simulink model "lga"  (R2020a)
settings: Solver=ode45  StartTime=0.0  StopTime=0.4  FixedStep=1e-6  MaxStep=0.04  RelTol=1e-3  EnableMultiTasking=on
PreLoadFcn:
  | power_13NodeTestFeeder_init;
values from neighbouring files (symbols this model uses):
  C_601 = [1.03835973183e-08  -3.28956213337e-09  -2.07596127216e-09; -3.28956213337e-09  9.8230300863e-09  -1.22250137004e-09; -2.07596127216e-09  -1.22250137004e-09  9.29377945947e-09]    [bus9.mat]    (also in matlab.mat)
  C_602 = [9.39333329896e-09  -1.78290377777e-09  -2.78635373607e-09; -1.78290377777e-09  8.5370713848e-09  -1.08586207709e-09; -2.78635373607e-09  -1.08586207709e-09  8.94105559107e-09]    [bus9.mat]    (also in matlab.mat)
  C_603 = [0  0  0; 0  7.76272711671e-09  -1.48325331387e-09; 0  -1.48325331387e-09  7.69036927641e-09]    [bus9.mat]    (also in matlab.mat)
  C_604 = [7.69036927641e-09  0  -1.48325331387e-09; 0  0  0; -1.48325331387e-09  0  7.76272711671e-09]    [bus9.mat]    (also in matlab.mat)
  C_605 = [0  0  0; 0  0  0; 0  0  7.44890176838e-09]    [bus9.mat]    (also in matlab.mat)
  C_606 = [1.59697709306e-07  -1.64824237567e-15  -1.64824237567e-15; -1.64824237567e-15  1.59697709306e-07  -1.64824237567e-15; -1.64824237567e-15  -1.64824237567e-15  1.59697709306e-07]    [bus9.mat]    (also in matlab.mat)
  C_607 = [1.46679066902e-07  0  0; 0  0  0; 0  0  0]    [bus9.mat]    (also in matlab.mat)
  ft2km = 0.0003048    [bus9.mat]    (also in matlab.mat)
  L_601 = [0.0016777459142  0.000826923199875  0.000698195470335; 0.000826923199875  0.00172702836123  0.000634408490396; 0.000698195470335  0.000634408490396  0.00170560121035]    [bus9.mat]    (also in matlab.mat)
  L_602 = [0.00194723354262  0.000698195470335  0.000826923199875; 0.000698195470335  0.00197508883877  0.000634408490396; 0.000826923199875  0.000634408490396  0.00199635116541]    [bus9.mat]    (also in matlab.mat)
  L_603 = [0  0  0; 0  0.00222034730427  0.000756708074671; 0  0.000756708074671  0.00223650007955]    [bus9.mat]    (also in matlab.mat)
  L_604 = [0.00223650007955  0  0.000756708074671; 0  0  0; 0.000756708074671  0  0.00222034730427]    [bus9.mat]    (also in matlab.mat)
  L_605 = [0  0  0; 0  0  0; 0  0  0.00222100660122]    [bus9.mat]    (also in matlab.mat)
  L_606 = [0.000735610572263  5.40623499221e-05  2.35698659721e-05; 5.40623499221e-05  0.000666054744009  5.40623499221e-05; 2.35698659721e-05  5.40623499221e-05  0.000735610572263]    [bus9.mat]    (also in matlab.mat)
  L_607 = [0.000844559393295  0  0; 0  0  0; 0  0  0]    [bus9.mat]    (also in matlab.mat)
  R_601 = [0.215305653249  0.0969341469174  0.0981768923907; 0.0969341469174  0.209713298619  0.0953807150757; 0.0981768923907  0.0953807150757  0.212136652292]    [bus9.mat]    (also in matlab.mat)
  R_602 = [0.467645121603  0.0981768923907  0.0969341469174; 0.0981768923907  0.464476120646  0.0953807150757; 0.0969341469174  0.0953807150757  0.462052766973]    [bus9.mat]    (also in matlab.mat)
  R_603 = [0  0  0; 0  0.826052916102  0.128375607392; 0  0.128375607392  0.822573228777]    [bus9.mat]    (also in matlab.mat)
  R_604 = [0.822573228777  0  0.128375607392; 0  0  0; 0.128375607392  0  0.826052916102]    [bus9.mat]    (also in matlab.mat)
  R_605 = [0  0  0; 0  0  0; 0  0  0.825928641555]    [bus9.mat]    (also in matlab.mat)
  R_606 = [0.495979718394  0.198342177539  0.177029092672; 0.198342177539  0.49032522649  0.198342177539; 0.177029092672  0.198342177539  0.495979718394]    [bus9.mat]    (also in matlab.mat)
  R_607 = [0.834192898952  0  0; 0  0  0; 0  0  0]    [bus9.mat]    (also in matlab.mat)
libraries: powerlib x54, powerlib_meascontrol x6
settings Model: Creator=MathWorks  LastModifiedBy=LMS Solution
settings DataIOCC: ExternalInput=getinputstruct(op_IEEE_13_node_5)  InitialState=getstatestruct(op_IEEE_13_node_5)  LimitDataPoints=on  SaveFormat=Array  SignalLoggingSaveFormat=ModelDataLogs  ReturnWorkspaceOutputs=off
settings OptimizationCC: ExpressionDepthLimit=2147483647  LifeSpan=inf
settings DebuggingCC: AlgebraicLoopMsg=none  UnderspecifiedInitializationDetection=Classic  MergeDetectMultiDrivingBlocksExec=none  FcnCallInpInsideContextMsg=warning  UnconnectedInputMsg=none  UnconnectedOutputMsg=none  UnconnectedLineMsg=none  AllowSymbolicDim=off  StateNameClashWarn=warning  SFUnexpectedBacktrackingDiag=warning  SFNoUnconditionalDefaultTransitionDiag=warning  SFExecutionAtInitializationDiag=none  ArithmeticOperatorsInVariantConditions=warning
settings HardwareCC: ProdBitPerPointer=32  ProdBitPerSizeT=32  ProdBitPerPtrDiffT=32  ProdLargestAtomicFloat=None  ProdIntDivRoundTo=Undefined  ProdEndianess=Unspecified  ProdWordSize=32  ProdHWDeviceType=32-bit Generic
settings ModelReferenceCC: PropagateSignalLabelsOutOfModel=off
settings SFSimCC: SimUseLocalCustomCode=off  CustomCodeUndefinedFunction=UseInterfaceOnly
settings RTWCC: RTWUseLocalCustomCode=off
settings CodeAppCC: StateflowObjectComments=on
settings GRTTargetCC: TargetLangStandard=C89/C90 (ANSI)  CombineOutputUpdateFcns=off  GRTInterface=on
settings ConfigComp: CovMetricSettings=dw  CovHtmlReporting=on  CovSaveCumulativeToWorkspaceVar=on  CovSaveSingleToWorkspaceVar=on  CovExternalEMLEnable=off  CovSFcnEnable=off
settings SimscapeCC: SimscapeNormalizeSystem=off

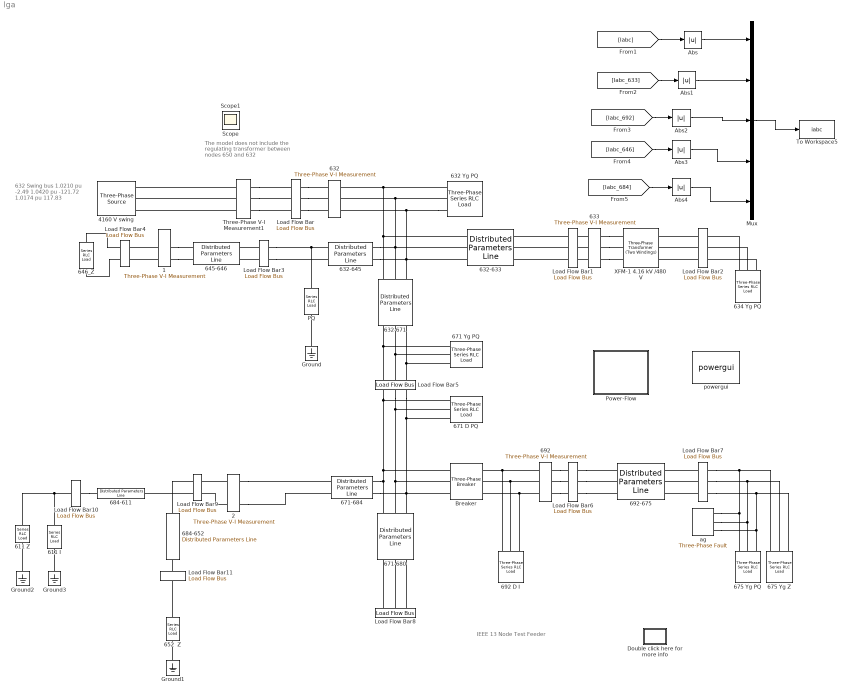
== system lga ==
  note: 632 Swing bus
      | 1.0210 pu -2.49
      | 1.0420 pu -121.72
      | 1.0174 pu 117.83
  note: IEEE 13 Node Test Feeder
  note: The model does not include
      | the regulating transformer
      | between nodes 650 and 632
  " 634 Yg PQ " : powerlib/Elements/Three-Phase Series RLC Load  LConnTagsString=A|B|C  Configuration=Y (grounded)  NominalVoltage=120e3  Vabc=[ 0.993805 1.0218 0.995862]*277.128  Vabcp=[1e3 1e3 1e3]  NominalFrequency=60  UnbalancedPower=on  ActivePower=1e+006  InductivePower=0  CapacitivePower=0  Pabc=[160 120 120]*1e3  QLabc=[110 90 90]*1e3  QCabc=[0 0 0]  Pabcp=[10e3 9e3 11e3]  QLabcp=[100 90 110]  QCabcp=[100 90 110]  Measurements=None  LoadType=constant PQ
      settings: SourceProductBaseCode=MT,PS
      settings: AttributesFormatString=|
      | P= %<Pabc> W
      | Ql=%<QLabc> var
      | Qc=%<QCabc> var
  1 : powerlib/Measurements/Three-Phase V-I Measurement  VoltageMeasurement=no  SetLabelV=on  LabelV=Vabc_646  Vpu=off  VpuLL=off  CurrentMeasurement=yes  SetLabelI=on  LabelI=Iabc_646  Ipu=off  Pbase=100e6  Vbase=4160  OutputType=Complex  PhasorSimulation=off  PSBequivalent=0
      settings: SourceProductBaseCode=MT,PS
  2 : powerlib/Measurements/Three-Phase V-I Measurement  VoltageMeasurement=no  SetLabelV=on  LabelV=Vabc_684  Vpu=off  VpuLL=off  CurrentMeasurement=yes  SetLabelI=on  LabelI=Iabc_684  Ipu=off  Pbase=100e6  Vbase=4160  OutputType=Complex  PhasorSimulation=off  PSBequivalent=0
      settings: SourceProductBaseCode=MT,PS
  4160 V swing : powerlib/Electrical Sources/Three-Phase Source  InternalConnection=Yg  VoltagePhases=on  Voltage=120e3  PhaseAngle=0  Voltage_phases=[ 1.021 1.042 1.0174]*2401.78  PhaseAngles_phases=[ -2.49 -121.72 117.83]  Frequency=60  NonIdealSource=off  SpecifyImpedance=on  Resistance=0.8929  Inductance=16.58e-3  ShortCircuitLevel=100e6  BaseVoltage=120e3  XRratio=10  BusType=swing  Pref=0  Qref=0  Prefabc=[0 0 0]  Qrefabc=[0 0 0]  Qmin="[-inf  -inf -inf]"  Qmax="[inf  inf inf]"
      settings: SourceProductBaseCode=MT,PS
  611 I : powerlib/Elements/Series RLC Load  LConnTagsString=a  RConnTagsString=__new0  NominalVoltage=0.986941*2401.78  NominalFrequency=60  ActivePower=170e3  InductivePower=80e3  CapacitivePower=0  Setx0=off  InitialVoltage=0  SetiL0=off  InitialCurrent=0  Measurements=Branch voltage and current  LoadType=constant I
      settings: SourceProductBaseCode=MT,PS
      settings: AttributesFormatString=|
      | P=%<ActivePower> W
      | Ql=%<InductivePower> var
      | Qc=%<CapacitivePower> var
  611 Z : powerlib/Elements/Series RLC Load  LConnTagsString=a  RConnTagsString=__new0  NominalVoltage=4160/sqrt(3)  NominalFrequency=60  ActivePower=0  InductivePower=0  CapacitivePower=100e3  Setx0=off  InitialVoltage=0  SetiL0=off  InitialCurrent=0  Measurements=None  LoadType=constant Z
      settings: SourceProductBaseCode=MT,PS
      settings: AttributesFormatString=|
      | P=%<ActivePower> W
      | Ql=%<InductivePower> var
      | Qc=%<CapacitivePower> var
  632 : powerlib/Measurements/Three-Phase V-I Measurement  VoltageMeasurement=phase-to-ground  SetLabelV=on  LabelV=Vabc_632  Vpu=off  VpuLL=off  CurrentMeasurement=yes  SetLabelI=on  LabelI=Iabc_632  Ipu=off  Pbase=100e6  Vbase=4160  OutputType=Complex  PhasorSimulation=off  PSBequivalent=0
      settings: SourceProductBaseCode=MT,PS
  632 Yg PQ : powerlib/Elements/Three-Phase Series RLC Load  LConnTagsString=A|B|C  Configuration=Y (grounded)  NominalVoltage=120e3  Vabc=[ 1.021 1.042 1.0174]*2401.78  Vabcp=[1e3 1e3 1e3]  NominalFrequency=60  UnbalancedPower=on  ActivePower=1e+006  InductivePower=0  CapacitivePower=0  Pabc="[17 66  117]*1e3/2"  QLabc="[10 38  68]*1e3/2"  QCabc=[0 0 0]  Pabcp=[10e3 9e3 11e3]  QLabcp=[100 90 110]  QCabcp=[100 90 110]  Measurements=None  LoadType=constant PQ
      settings: SourceProductBaseCode=MT,PS
      settings: AttributesFormatString=|
      | P= %<Pabc> W
      | Ql=%<QLabc> var
      | Qc=%<QCabc> var
  632-633 : powerlib/Elements/Distributed Parameters Line  Phases=3  Frequency=60  Resistance=R_602  Inductance=L_602  Capacitance=C_602  Length=500*ft2km  x1=[501.293872949305 4241.45382070984 4282.1906180408;376.991118430775 376.991118430775 376.991118430775;-2.26141264082395 -0.341585700927958 -1.91682015260342]  x2=[504.561752510722 4230.83532883347 4271.81237473623;376.991118430775 376.991118430775 376.991118430775;-2.26353818089954 -0.342283942523961 -1.91743130559756]  x3=[16.6662219254557 117.159865311925 102.981784246328;376.991118430775 376.991118430775 376.991118430775;2.64824122421638 2.14567196099075 0.446243240990135]  x4=[16.4574042983544 140.145540779761 120.267032711561;376.991118430775 376.991118430775 376.991118430775;-0.571833890760735 -0.875489993465733 -2.56205104695807]  x5=6.41053351781503e-07  V1=ones(3,3)  V2=ones(3,3)  I1=ones(3,3)  I2=ones(3,3)  nHarmo=1  Measurements=None
      settings: SourceProductBaseCode=MT,PS
  632-645 : powerlib/Elements/Distributed Parameters Line  Phases=2  Frequency=60  Resistance=R_603(2:3,2:3)  Inductance=L_603(2:3,2:3)  Capacitance=C_603(2:3,2:3)  Length=500*ft2km  x1=[4264.5022731202 2449.41675834518;376.991118430775 376.991118430775;-1.6135259286109 3.12258289264097]  x2=[4292.22338635442 2455.21000720595;376.991118430775 376.991118430775;-1.61412234121454 3.12992995046501]  x3=[213.164870940156 87.6157732608083;376.991118430775 376.991118430775;-2.34395632993981 -2.78111404185977]  x4=[197.723678038707 81.051948801637;376.991118430775 376.991118430775;0.725343758835368 0.39265291515961]  x5=6.57914367465262e-07  V1=ones(3,3)  V2=ones(3,3)  I1=ones(3,3)  I2=ones(3,3)  nHarmo=1  Measurements=None
      settings: SourceProductBaseCode=MT,PS
  632-671 : powerlib/Elements/Distributed Parameters Line  Phases=3  Frequency=60  Resistance=R_601  Inductance=L_601  Capacitance=C_601  Length=2000*ft2km  x1=[411.258730357127 4262.40190274633 4279.48776495495;376.991118430775 376.991118430775 376.991118430775;2.58884794833249 0.275840323894815 1.83440828309495]  x2=[347.306680493627 4150.58183459432 4225.17464338496;376.991118430775 376.991118430775 376.991118430775;2.89593582452205 0.256745851928195 1.79323964699828]  x3=[175.735197365501 639.164110681117 682.76866552397;376.991118430775 376.991118430775 376.991118430775;-2.71340597147986 2.78575301834637 -1.35887211837434]  x4=[175.070217002063 666.480663073621 708.955927243058;376.991118430775 376.991118430775 376.991118430775;0.432442150729287 -0.326762390577467 1.78386018236244]  x5=2.51909782126786e-06  V1=ones(3,3)  V2=ones(3,3)  I1=ones(3,3)  I2=ones(3,3)  nHarmo=1  Measurements=None
      settings: SourceProductBaseCode=MT,PS
  633 : powerlib/Measurements/Three-Phase V-I Measurement  VoltageMeasurement=phase-to-ground  SetLabelV=on  LabelV=Vabc_633  Vpu=off  VpuLL=off  CurrentMeasurement=yes  SetLabelI=on  LabelI=Iabc_633  Ipu=off  Pbase=100e6  Vbase=4160  OutputType=Complex  PhasorSimulation=off  PSBequivalent=0
      settings: SourceProductBaseCode=MT,PS
  645-646 : powerlib/Elements/Distributed Parameters Line  Phases=2  Frequency=60  Resistance=R_603(2:3,2:3)  Inductance=L_603(2:3,2:3)  Capacitance=C_603(2:3,2:3)  Length=300*ft2km  x1=[4254.01788248819 2449.39386138164;376.991118430775 376.991118430775;-1.61382385460359 3.12270982637929]  x2=[4264.5022731202 2449.41675834518;376.991118430775 376.991118430775;-1.6134413207014 3.12268210379026]  x3=[139.790624472069 3.30345191812981;376.991118430775 376.991118430775;-2.09472435821047 2.98426093088177]  x4=[121.290812771644 3.84897379292667;376.991118430775 376.991118430775;0.96544378333039 -3.04191355544302]  x5=3.94748620479157e-07  V1=ones(3,3)  V2=ones(3,3)  I1=ones(3,3)  I2=ones(3,3)  nHarmo=1  Measurements=None
      settings: SourceProductBaseCode=MT,PS
  646_Z : powerlib/Elements/Series RLC Load  LConnTagsString=a  RConnTagsString=__new0  NominalVoltage=4160  NominalFrequency=60  ActivePower=230e3  InductivePower=132e3  CapacitivePower=0  Setx0=off  InitialVoltage=0  SetiL0=off  InitialCurrent=0  Measurements=None  LoadType=constant Z
      settings: SourceProductBaseCode=MT,PS
      settings: AttributesFormatString=|
      | P=%<ActivePower> W
      | Ql=%<InductivePower> var
      | Qc=%<CapacitivePower> var
  "652  Z " : powerlib/Elements/Series RLC Load  LConnTagsString=a  RConnTagsString=__new0  NominalVoltage=4160/sqrt(3)  NominalFrequency=60  ActivePower=128e3  InductivePower=86e3  CapacitivePower=0  Setx0=off  InitialVoltage=0  SetiL0=off  InitialCurrent=0  Measurements=None  LoadType=constant Z
      settings: SourceProductBaseCode=MT,PS
      settings: AttributesFormatString=|
      | P=%<ActivePower> W
      | Ql=%<InductivePower> var
      | Qc=%<CapacitivePower> var
  671 D PQ : powerlib/Elements/Three-Phase Series RLC Load  LConnTagsString=A|B|C  Configuration=Delta  NominalVoltage=120e3  Vabc="[1  1  1]*120e3/sqrt(3)"  Vabcp=[ 1.73773 1.77224 1.71484]*2401.78  NominalFrequency=60  UnbalancedPower=on  ActivePower=1e+006  InductivePower=0  CapacitivePower=0  Pabc="[17 66  117]*1e3/2"  QLabc="[10 38  68]*1e3/2"  QCabc=[0 0 0]  Pabcp=[385 385 385 ]*1e3  QLabcp=[220 220 220]*1e3  QCabcp="[0  0  0]"  Measurements=Branch voltages and currents  LoadType=constant PQ
      settings: SourceProductBaseCode=MT,PS
      settings: AttributesFormatString=|
      | P= %<Pabcp> W
      | Ql=%<QLabcp> var
      | Qc=%<QCabcp> var
  671 Yg PQ : powerlib/Elements/Three-Phase Series RLC Load  LConnTagsString=A|B|C  Configuration=Y (grounded)  NominalVoltage=120e3  Vabc=[ 0.987076 1.0519 0.978043]*2401.78  Vabcp=[1e3 1e3 1e3]  NominalFrequency=60  UnbalancedPower=on  ActivePower=1e+006  InductivePower=0  CapacitivePower=0  Pabc="[17 66  117]*1e3/2"  QLabc="[10 38  68]*1e3/2"  QCabc=[0 0 0]  Pabcp=[10e3 9e3 11e3]  QLabcp=[100 90 110]  QCabcp=[100 90 110]  Measurements=None  LoadType=constant PQ
      settings: SourceProductBaseCode=MT,PS
      settings: AttributesFormatString=|
      | P= %<Pabc> W
      | Ql=%<QLabc> var
      | Qc=%<QCabc> var
  671-680 : powerlib/Elements/Distributed Parameters Line  Phases=3  Frequency=60  Resistance=R_601  Inductance=L_601  Capacitance=C_601  Length=1000*ft2km  x1=[347.306680493627 4150.58183459432 4225.17464338496;376.991118430775 376.991118430775 376.991118430775;2.89641066327458 0.257138768490046 1.79363062709424]  x2=[347.306719647812 4150.58215498482 4225.17496632654;376.991118430775 376.991118430775 376.991118430775;2.89641062451109 0.257138741099331 1.79363060588642]  x3=[0.463161645569061 16.4122452656798 13.019790636799;376.991118430775 376.991118430775 376.991118430775;2.89593580408531 0.256745838252545 1.79323963640573]  x4=[0.463161644447677 16.4122452662158 13.0197906368517;376.991118430775 376.991118430775 376.991118430775;2.89641062556775 0.257138741079497 1.79363060587495]  x5=1.25954891063393e-06  V1=ones(3,3)  V2=ones(3,3)  I1=ones(3,3)  I2=ones(3,3)  nHarmo=1  Measurements=None
      settings: SourceProductBaseCode=MT,PS
  671-684 : powerlib/Elements/Distributed Parameters Line  Phases=2  Frequency=60  Resistance=R_604([1 3],[1 3])  Inductance=L_604([1 3],[1 3])  Capacitance=C_604([1 3],[1 3])  Length=300*ft2km  x1=[2313.59941272332 4108.10470701944;376.991118430775 376.991118430775;0.955996647177928 2.53692176309295]  x2=[2315.45218770047 4117.95026948363;376.991118430775 376.991118430775;0.957119003354268 2.53797965056326]  x3=[27.0373603664756 142.306206395117;376.991118430775 376.991118430775;1.02915892801391 2.29887293502492]  x4=[20.3577083958235 122.39660260244;376.991118430775 376.991118430775;-2.08852277525659 -0.882473110536219]  x5=3.94748620479157e-07  V1=ones(3,3)  V2=ones(3,3)  I1=ones(3,3)  I2=ones(3,3)  nHarmo=1  Measurements=None
      settings: SourceProductBaseCode=MT,PS
  675 Yg PQ : powerlib/Elements/Three-Phase Series RLC Load  LConnTagsString=A|B|C  Configuration=Y (grounded)  NominalVoltage=120e3  Vabc=[ 0.98063 1.05431 0.975983]*2401.78  Vabcp=[1e3 1e3 1e3]  NominalFrequency=60  UnbalancedPower=on  ActivePower=1e+006  InductivePower=0  CapacitivePower=0  Pabc="[485  68  290]*1e3"  QLabc="[190  60  212]*1e3"  QCabc=[0 0 0]  Pabcp=[10e3 9e3 11e3]  QLabcp=[100 90 110]  QCabcp=[100 90 110]  Measurements=Branch voltages and currents  LoadType=constant PQ
      settings: SourceProductBaseCode=MT,PS
      settings: AttributesFormatString=|
      | P= %<Pabc> W
      | Ql=%<QLabc> var
      | Qc=%<QCabc> var
  675 Yg Z : powerlib/Elements/Three-Phase Series RLC Load  LConnTagsString=A|B|C  Configuration=Y (grounded)  NominalVoltage=120e3  Vabc="[1  1  1]*4160/sqrt(3)"  Vabcp=[1e3 1e3 1e3]  NominalFrequency=60  UnbalancedPower=on  ActivePower=1e+006  InductivePower=0  CapacitivePower=0  Pabc=[0 0 0]  QLabc=[0 0 0]  QCabc=[200 200 200]*1e3  Pabcp=[10e3 9e3 11e3]  QLabcp=[100 90 110]  QCabcp=[100 90 110]  Measurements=None  LoadType=constant Z
      settings: SourceProductBaseCode=MT,PS
      settings: AttributesFormatString=|
      | P= %<Pabc> W
      | Ql=%<QLabc> var
      | Qc=%<QCabc> var
  684-611 : powerlib/Elements/Distributed Parameters Line  Phases=1  Frequency=60  Resistance=R_605(3,3)  Inductance=L_605(3,3)  Capacitance=C_605(3,3)  Length=300*ft2km  x1=[3308.40125911969;376.991118430775;2.0202288607597]  x2=[3315.18688864096;376.991118430775;2.02277401911421]  x3=[106.641161603485;376.991118430775;2.11647233822245]  x4=[94.5740657861888;376.991118430775;-1.01294980309294]  x5=3.71926621942778e-07  V1=ones(3,3)  V2=ones(3,3)  I1=ones(3,3)  I2=ones(3,3)  nHarmo=1  Measurements=None
      settings: SourceProductBaseCode=MT,PS
  684-652 : powerlib/Elements/Distributed Parameters Line  Phases=1  Frequency=60  Resistance=R_607(1,1)  Inductance=L_607(1,1)  Capacitance=C_607(1,1)  Length=800*ft2km  x1=[3355.37633628676;376.991118430775;-0.0936238783207487]  x2=[3336.4536414072;376.991118430775;-0.0923228877162377]  x3=[57.8438476752768;376.991118430775;2.01984537128709]  x4=[127.863153778251;376.991118430775;-0.49132566875403]  x5=2.71396421650751e-06  V1=ones(3,3)  V2=ones(3,3)  I1=ones(3,3)  I2=ones(3,3)  nHarmo=1  Measurements=None
      settings: SourceProductBaseCode=MT,PS
  692 : powerlib/Measurements/Three-Phase V-I Measurement  VoltageMeasurement=phase-to-ground  SetLabelV=on  LabelV=Vabc_692  Vpu=off  VpuLL=off  CurrentMeasurement=yes  SetLabelI=on  LabelI=Iabc_692  Ipu=off  Pbase=100e6  Vbase=4160  OutputType=Complex  PhasorSimulation=off  PSBequivalent=0
      settings: SourceProductBaseCode=MT,PS
  692 D I : powerlib/Elements/Three-Phase Series RLC Load  LConnTagsString=A|B|C  Configuration=Delta  NominalVoltage=120e3  Vabc="[1  1  1]*120e3/sqrt(3)"  Vabcp=[ 1.73488 1.75203 1.72341]*2401.78  NominalFrequency=60  UnbalancedPower=on  ActivePower=1e+006  InductivePower=0  CapacitivePower=0  Pabc="[17 66  117]*1e3/2"  QLabc="[10 38  68]*1e3/2"  QCabc=[0 0 0]  Pabcp=[1e-6 1e-6 170 ]*1e3  QLabcp=[0 0 151]*1e3  QCabcp="[0  0  0]"  Measurements=Branch voltages and currents  LoadType=constant I
      settings: SourceProductBaseCode=MT,PS
      settings: AttributesFormatString=|
      | P= %<Pabcp> W
      | Ql=%<QLabcp> var
      | Qc=%<QCabcp> var
  692-675 : powerlib/Elements/Distributed Parameters Line  Phases=3  Frequency=60  Resistance=R_606  Inductance=L_606  Capacitance=C_606  Length=500*ft2km  x1=[241.946426527935 4119.38081603559 4253.12123917423;376.991118430775 376.991118430775 376.991118430775;-1.73462308165995 -0.601802873673824 -2.15225057055155]  x2=[257.258395716564 4106.92718949573 4248.47317831092;376.991118430775 376.991118430775 376.991118430775;-1.8050627630111 -0.605002039585924 -2.15361016422562]  x3=[166.085012520769 223.901518079614 66.0340850301017;376.991118430775 376.991118430775 376.991118430775;-2.93628354257307 2.68229298009573 1.40461019515309]  x4=[163.433093099822 346.203759262503 198.017412027977;376.991118430775 376.991118430775 376.991118430775;0.165702552369017 -0.510503131256597 -2.01797432719262]  x5=1.72234634931087e-06  V1=ones(3,3)  V2=ones(3,3)  I1=ones(3,3)  I2=ones(3,3)  nHarmo=1  Measurements=None
      settings: SourceProductBaseCode=MT,PS
  Abs{,1..4} (5 alike) : Abs
  Breaker : powerlib/Elements/Three-Phase Breaker  InitialState=closed  SwitchA=off  SwitchB=off  SwitchC=off  SwitchTimes=[0.5 ]  External=off  BreakerResistance=0.0001  SnubberResistance=inf  SnubberCapacitance=0  Measurements=None
      settings: SourceProductBaseCode=MT,PS
  Double click here for more info : Subsystem
      settings: OpenFcn=showdemo(bdroot(gcb))
      mask Display: disp('?')
  Ground{,1..3} (4 alike) : powerlib/Elements/Ground  LConnTagsString=a
      settings: SourceProductBaseCode=MT,PS
  Load Flow Bar : powerlib/Measurements/Load Flow Bus  LConnTagsString=a|b|c  RConnTagsString=a|b|c  Phases=ABC  Connectors=on both sides  ID=632  Vbase=4160/sqrt(3)  Vref="[ 1.0210  1.0420  1.0174]"  Vangle="[ -2.49  -121.72  117.83]"  VLF=1.021  VLFb=1.042  VLFc=1.017  angleLF=-2.49  angleLFb=-121.7  angleLFc=117.8
      settings: AttributesFormatString=%<ID>  SourceProductBaseCode=MT,PS
  Load Flow Bar1 : powerlib/Measurements/Load Flow Bus  LConnTagsString=a|b|c  RConnTagsString=a|b|c  Phases=ABC  Connectors=on both sides  ID=633  Vbase=4160/sqrt(3)  Vref=[1.0 1.0 1.0]  Vangle=[0 -120 120]  VLF=1.018  VLFb=1.04  VLFc=1.015  angleLF=-2.559  angleLFb=-121.8  angleLFc=117.8
      settings: AttributesFormatString=%<ID>  SourceProductBaseCode=MT,PS
  Load Flow Bar10 : powerlib/Measurements/Load Flow Bus  LConnTagsString=a  RConnTagsString=a  Phases=C  Connectors=on both sides  ID=611  Vbase=4160/sqrt(3)  Vref=1.0  Vangle=0  VLF=NaN  VLFb=NaN  VLFc=0.9741  angleLF=NaN  angleLFb=NaN  angleLFc=115.8
      settings: AttributesFormatString=%<ID>  SourceProductBaseCode=MT,PS
  Load Flow Bar11 : powerlib/Measurements/Load Flow Bus  LConnTagsString=a  RConnTagsString=a  Phases=A  Connectors=on both sides  ID=652  Vbase=4160/sqrt(3)  Vref=1.0  Vangle=0  VLF=0.9796  VLFb=NaN  VLFc=NaN  angleLF=-5.477  angleLFb=NaN  angleLFc=NaN
      settings: AttributesFormatString=%<ID>  SourceProductBaseCode=MT,PS
  Load Flow Bar2 : powerlib/Measurements/Load Flow Bus  LConnTagsString=a|b|c  RConnTagsString=a|b|c  Phases=ABC  Connectors=on both sides  ID=634  Vbase=480/sqrt(3)  Vref=[1.0 1.0 1.0]  Vangle=[0 -120 120]  VLF=0.9938  VLFb=1.022  VLFc=0.9959  angleLF=-3.236  angleLFb=-122.2  angleLFc=117.4
      settings: AttributesFormatString=%<ID>  SourceProductBaseCode=MT,PS
  Load Flow Bar3 : powerlib/Measurements/Load Flow Bus  LConnTagsString=a|b  RConnTagsString=a|b  Phases=BC  Connectors=on both sides  ID=645  Vbase=4160/sqrt(3)  Vref=[1.0 1.0 ]  Vangle=[0 0]  VLF=NaN  VLFb=1.033  VLFc=1.015  angleLF=NaN  angleLFb=-121.9  angleLFc=117.9
      settings: AttributesFormatString=%<ID>  SourceProductBaseCode=MT,PS
  Load Flow Bar4 : powerlib/Measurements/Load Flow Bus  LConnTagsString=a|b  RConnTagsString=a|b  Phases=BC  Connectors=on both sides  ID=646  Vbase=4160/sqrt(3)  Vref=[1.0 1.0 ]  Vangle=[0 0]  VLF=NaN  VLFb=1.031  VLFc=1.013  angleLF=NaN  angleLFb=-122  angleLFc=117.9
      settings: AttributesFormatString=%<ID>  SourceProductBaseCode=MT,PS
  Load Flow Bar5 : powerlib/Measurements/Load Flow Bus  LConnTagsString=a|b|c  RConnTagsString=a|b|c  Phases=ABC  Connectors=on both sides  ID=671  Vbase=4160/sqrt(3)  Vref=[1.0 1.0 1.0]  Vangle=[0 -120 120]  VLF=0.9871  VLFb=1.052  VLFc=0.978  angleLF=-5.529  angleLFb=-122.4  angleLFc=116
      settings: AttributesFormatString=%<ID>  SourceProductBaseCode=MT,PS
  Load Flow Bar6 : powerlib/Measurements/Load Flow Bus  LConnTagsString=a|b|c  RConnTagsString=a|b|c  Phases=ABC  Connectors=on both sides  ID=692  Vbase=4160/sqrt(3)  Vref=[1.0 1.0 1.0]  Vangle=[0 -120 120]  VLF=0.9871  VLFb=1.052  VLFc=0.978  angleLF=-5.528  angleLFb=-122.4  angleLFc=116
      settings: AttributesFormatString=%<ID>  SourceProductBaseCode=MT,PS
  Load Flow Bar7 : powerlib/Measurements/Load Flow Bus  LConnTagsString=a|b|c  RConnTagsString=a|b|c  Phases=ABC  Connectors=on both sides  ID=675  Vbase=4160/sqrt(3)  Vref=[1.0 1.0 1.0]  Vangle=[0 -120 120]  VLF=0.9806  VLFb=1.054  VLFc=0.976  angleLF=-5.774  angleLFb=-122.6  angleLFc=116
      settings: AttributesFormatString=%<ID>  SourceProductBaseCode=MT,PS
  Load Flow Bar8 : powerlib/Measurements/Load Flow Bus  LConnTagsString=a|b|c  Phases=ABC  Connectors=on one side  ID=680  Vbase=4160/sqrt(3)  Vref=[1.0 1.0 1.0]  Vangle=[0 -120 120]  VLF=0.9871  VLFb=1.052  VLFc=0.978  angleLF=-5.529  angleLFb=-122.4  angleLFc=116
      settings: AttributesFormatString=%<ID>  SourceProductBaseCode=MT,PS
  Load Flow Bar9 : powerlib/Measurements/Load Flow Bus  LConnTagsString=a|b  RConnTagsString=a|b  Phases=AC  Connectors=on both sides  ID=684  Vbase=4160/sqrt(3)  Vref=[1.0 1.0 ]  Vangle=[0 -120 ]  VLF=0.9851  VLFb=NaN  VLFc=0.9761  angleLF=-5.551  angleLFb=NaN  angleLFc=115.9
      settings: AttributesFormatString=%<ID>  SourceProductBaseCode=MT,PS
  Mux : Mux  Inputs=5
  PQ : powerlib/Elements/Series RLC Load  LConnTagsString=a  RConnTagsString=__new0  NominalVoltage=1.03289*2401.78  NominalFrequency=60  ActivePower=170e3  InductivePower=125e3  CapacitivePower=0  Setx0=off  InitialVoltage=0  SetiL0=off  InitialCurrent=0  Measurements=None  LoadType=constant PQ
      settings: SourceProductBaseCode=MT,PS
      settings: AttributesFormatString=|
      | P=%<ActivePower> W
      | Ql=%<InductivePower> var
      | Qc=%<CapacitivePower> var
  Power-Flow : Subsystem
      mask Display: disp('Power-Flow\nResults')
  Three-Phase V-I Measurement1 : powerlib/Measurements/Three-Phase V-I Measurement  VoltageMeasurement=phase-to-ground  SetLabelV=on  LabelV=Vabc  Vpu=off  VpuLL=off  CurrentMeasurement=yes  SetLabelI=on  LabelI=Iabc  Ipu=on  Pbase=1e6  Vbase=4160  OutputType=Complex  PhasorSimulation=off  PSBequivalent=0
  To Workspace5 : ToWorkspace  VariableName=iabc  SampleTime=-1
      settings: MaxDataPoints=10
  XFM-1 4.16 kV /480 V : powerlib/Elements/Three-Phase Transformer (Two Windings)  Winding1Connection=Yg  Winding2Connection=Yg  CoreType=Three single-phase transformers  SetSaturation=off  Hysteresis=off  DataFile='hysteresis'  SetInitialFlux=off  Measurements=None  UNITS=pu  NominalPower=[ 500e3 , 60 ]  Winding1=[4160 0.011 0.02]  Winding2=[480 0 0]  Rm=500  Lm=500  L0=0.5  Saturation=[0 0;0.0024 1.2;1 1.52]  InitialFluxes=[0.8 -0.8 0.7]  BreakLoop=off  DiscreteSolver=Trapezoidal iterative  DataType=off  TransfoNumber=1
      settings: SourceProductBaseCode=MT,PS
  ag : powerlib/Elements/Three-Phase Fault  InitialStates=0  FaultA=on  FaultB=off  FaultC=off  GroundFault=on  SwitchTimes=[0.2 0.4]  External=off  SwitchStatus=NaN  FaultResistance=0.01  GroundResistance=0.01  SnubberResistance=1e6  SnubberCapacitance=inf  Measurements=None
  powergui : powerlib/powergui  Priority=1  SimulationMode=Discrete phasor  SampleTime=0.004  frequency=60  Iterations=50  frequencyindice=60  Pbase=100e3  ErrMax=0.0001  UnitsV=kV  UnitsW=kW  buscounter=0  FunctionMessages=off  echomessages=off  EnableUseOfTLC=off  CurrentSourceSwitches=off  DisableSnubberDevices=off  DisableRonSwitches=off  DisableVfSwitches=off  DisplayEquations=off  AutomaticDiscreteSolvers=off  SolverType=Tustin/Backward Euler (TBE)  Interpol=off  ExternalGateDelay=off  methode=off  Ts=0  x0status=blocks  SPID=off  SwTol=0  HookPort=off  NonlinearTolerance=1e-4  nMaxIteration=100  ContinueOnMaxIteration=off  RestoreLinks=warning  ResistiveCurrentMeasurement=off  Frange=[0:2:500]  Ylog=off  Xlog=on  ShowGrid=off  save=off  variable=ZData  structure=0  ZoomFFT=on  StartTime=0.0  cycles=1  DisplayStyle=1  fundamental=60  FreqAxis=off  MaxFrequency=1000  frequencyindicesteady=1  RmsSteady=1  display=off
  Scope : Scope
  Scope1 : Scope
  wires:
  Abs2/1 -> Mux/3
  [Iabc_633] -> Abs1/1
  Abs1/1 -> Mux/2
  Mux/1 -> To Workspace5/1
  [Iabc] -> Abs/1
  Abs/1 -> Mux/1
  [Iabc_692] -> Abs2/1
  [Iabc_646] -> Abs3/1
  [Iabc_684] -> Abs4/1
  Abs3/1 -> Mux/4
  Abs4/1 -> Mux/5
  connections:
  Load Flow Bar5/LConn2 -- 632-671/RConn2 -- 671 Yg PQ/LConn2
  Load Flow Bar5/LConn1 -- 632-671/RConn1 -- 671 Yg PQ/LConn1
  Load Flow Bar5/LConn3 -- 671 Yg PQ/LConn3 -- 632-671/RConn3
  Load Flow Bar7/LConn1 -- ag/LConn1 -- 675 Yg PQ/LConn1 -- 675 Yg Z/LConn1
  Load Flow Bar7/LConn2 -- ag/LConn2 -- 675 Yg PQ/LConn2 -- 675 Yg Z/LConn2
  Load Flow Bar7/LConn3 -- ag/LConn3 -- 675 Yg PQ/LConn3 -- 675 Yg Z/LConn3
  Load Flow Bar7/RConn1 -- 692-675/RConn1
  Load Flow Bar8/LConn1 -- 671-680/RConn1
  Load Flow Bar8/LConn3 -- 671-680/RConn3
  Load Flow Bar7/RConn3 -- 692-675/RConn3
  Load Flow Bar7/RConn2 -- 692-675/RConn2
  Load Flow Bar8/LConn2 -- 671-680/RConn2
  Load Flow Bar10/RConn1 -- 684-611/LConn1
  Load Flow Bar1/LConn1 -- 632-633/RConn1
  Load Flow Bar1/LConn2 -- 632-633/RConn2
  Load Flow Bar1/LConn3 -- 632-633/RConn3
  Load Flow Bar2/LConn1 -- XFM-1 4.16 kV /480 V/RConn1
  Load Flow Bar2/LConn2 -- XFM-1 4.16 kV /480 V/RConn2
  Load Flow Bar2/LConn3 -- XFM-1 4.16 kV /480 V/RConn3
  Load Flow Bar3/RConn1 -- PQ/LConn1 -- 632-645/LConn1
  Load Flow Bar3/RConn2 -- 632-645/LConn2
  Load Flow Bar3/LConn1 -- 645-646/RConn1
  Load Flow Bar3/LConn2 -- 645-646/RConn2
  Load Flow Bar6/LConn1 -- 692-675/LConn1
  Load Flow Bar6/LConn2 -- 692-675/LConn2
  Load Flow Bar6/LConn3 -- 692-675/LConn3
  671 D PQ/LConn1 -- Breaker/LConn1 -- 671-684/RConn1 -- 671-680/LConn1 -- Load Flow Bar5/RConn1
  671 D PQ/LConn2 -- Load Flow Bar5/RConn2 -- Breaker/LConn2 -- 671-680/LConn2
  671-680/LConn3 -- 671-684/RConn2 -- Breaker/LConn3 -- 671 D PQ/LConn3 -- Load Flow Bar5/RConn3
  692 D I/LConn1 -- 692/LConn1 -- Breaker/RConn1
  692 D I/LConn2 -- 692/LConn2 -- Breaker/RConn2
  692 D I/LConn3 -- 692/LConn3 -- Breaker/RConn3
  Load Flow Bar11/LConn1 -- 684-652/RConn1
  "652  Z "/LConn1 -- Load Flow Bar11/RConn1
  Load Flow Bar9/LConn2 -- 684-611/RConn1
  Load Flow Bar9/LConn1 -- 684-652/LConn1
  " 634 Yg PQ "/LConn1 -- Load Flow Bar2/RConn1
  " 634 Yg PQ "/LConn2 -- Load Flow Bar2/RConn2
  " 634 Yg PQ "/LConn3 -- Load Flow Bar2/RConn3
  Ground/LConn1 -- PQ/RConn1
  646_Z/LConn1 -- Load Flow Bar4/LConn1
  Load Flow Bar4/LConn2 -- 646_Z/RConn1
  Ground2/LConn1 -- 611 Z/RConn1
  611 Z/LConn1 -- 611 I/LConn1 -- Load Flow Bar10/LConn1
  Ground1/LConn1 -- "652  Z "/RConn1
  Ground3/LConn1 -- 611 I/RConn1
  692/RConn1 -- Load Flow Bar6/RConn1
  692/RConn2 -- Load Flow Bar6/RConn2
  692/RConn3 -- Load Flow Bar6/RConn3
  633/LConn1 -- Load Flow Bar1/RConn1
  633/LConn2 -- Load Flow Bar1/RConn2
  633/LConn3 -- Load Flow Bar1/RConn3
  633/RConn3 -- XFM-1 4.16 kV /480 V/LConn3
  633/RConn2 -- XFM-1 4.16 kV /480 V/LConn2
  633/RConn1 -- XFM-1 4.16 kV /480 V/LConn1
  Load Flow Bar/RConn1 -- 632/LConn1
  Load Flow Bar/RConn2 -- 632/LConn2
  Load Flow Bar/RConn3 -- 632/LConn3
  632 Yg PQ/LConn1 -- 632-671/LConn1 -- 632-633/LConn1 -- 632/RConn1
  632 Yg PQ/LConn2 -- 632/RConn2 -- 632-671/LConn2 -- 632-645/RConn1 -- 632-633/LConn2
  632 Yg PQ/LConn3 -- 632-671/LConn3 -- 632-645/RConn2 -- 632-633/LConn3 -- 632/RConn3
  Three-Phase V-I Measurement1/LConn1 -- 4160 V swing/RConn1
  Three-Phase V-I Measurement1/LConn2 -- 4160 V swing/RConn2
  Three-Phase V-I Measurement1/LConn3 -- 4160 V swing/RConn3
  Three-Phase V-I Measurement1/RConn1 -- Load Flow Bar/LConn1
  Three-Phase V-I Measurement1/RConn2 -- Load Flow Bar/LConn2
  Three-Phase V-I Measurement1/RConn3 -- Load Flow Bar/LConn3
  1/LConn2 -- Load Flow Bar4/RConn1
  1/LConn3 -- Load Flow Bar4/RConn2
  1/RConn2 -- 645-646/LConn1
  1/RConn3 -- 645-646/LConn2
  2/LConn1 -- Load Flow Bar9/RConn1
  2/RConn1 -- 671-684/LConn1
  2/LConn3 -- Load Flow Bar9/RConn2
  2/RConn3 -- 671-684/LConn2

== system lga/Double click here for more info ==

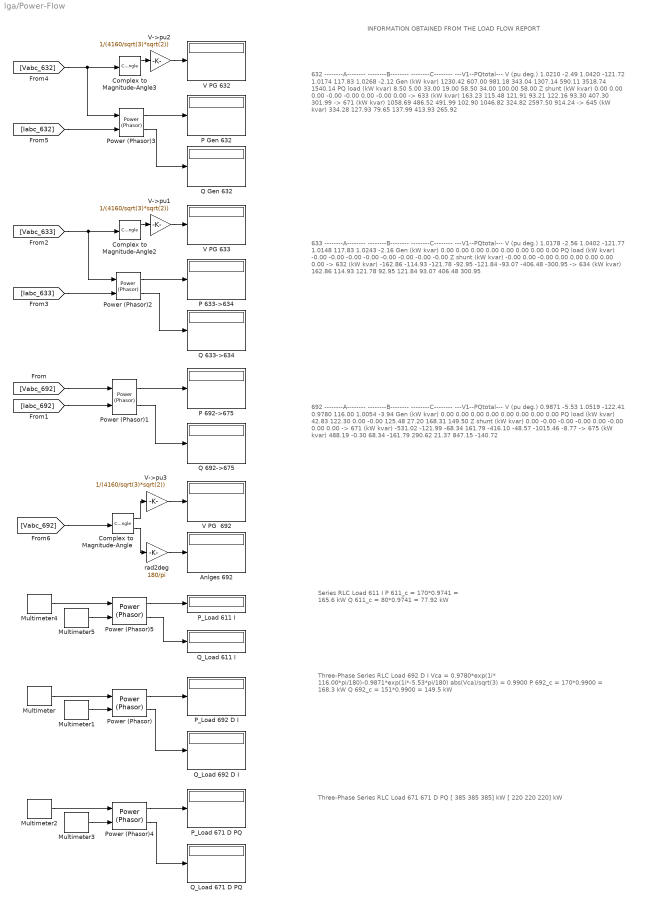
== system lga/Power-Flow ==
  note: INFORMATION OBTAINED FROM THE LOAD FLOW REPORT
  note: Series RLC Load 611 I
      | P 611_c = 170*0.9741 = 165.6 kW
      | Q 611_c = 80*0.9741 = 77.92 kW
  note: Three-Phase Series RLC Load 692 D I
      | Vca = 0.9780*exp(1i* 116.00*pi/180)-0.9871*exp(1i*-5.53*pi/180)
      | abs(Vca)/sqrt(3) = 0.9900
      | P 692_c = 170*0.9900 = 168.3 kW
      | Q 692_c = 151*0.9900 = 149.5 kW
  note: Three-Phase Series RLC Load 671 671 D PQ
      | [ 385 385 385] kW
      | [ 220 220 220] kW
  note: 632 --------A-------- --------B-------- --------C-------- ---V1--PQtotal---
      | V (pu deg.) 1.0210 -2.49 1.0420 -121.72 1.0174 117.83 1.0268 -2.12
      | Gen (kW kvar) 1230.42 607.00 981.18 343.04 1307.14 590.11 3518.74 1540.14
      | PQ load (kW kvar) 8.50 5.00 33.00 19.00 58.50 34.00 100.00 58.00
      | Z shunt (kW kvar) 0.00 0.00 0.00 -0.00 -0.00 0.00 -0.00 0.00
      |
      | -> 633 (kW kvar) 163.23 115.48 121.91 93.21 122.16 93.30 407.30 301.99
      | -> 671 (kW kvar) 1058.69 486.52 491.99 102.90 1046.82 324.82 2597.50 914.24
      | -> 645 (kW kvar) 334.28 127.93 79.65 137.99 413.93 265.92
  note: 633 --------A-------- --------B-------- --------C-------- ---V1--PQtotal---
      | V (pu deg.) 1.0178 -2.56 1.0402 -121.77 1.0148 117.83 1.0243 -2.16
      | Gen (kW kvar) 0.00 0.00 0.00 0.00 0.00 0.00 0.00 0.00
      | PQ load (kW kvar) -0.00 -0.00 -0.00 -0.00 -0.00 -0.00 -0.00 -0.00
      | Z shunt (kW kvar) -0.00 0.00 -0.00 0.00 0.00 0.00 0.00 0.00
      |
      | -> 632 (kW kvar) -162.86 -114.93 -121.78 -92.95 -121.84 -93.07 -406.48 -300.95
      | -> 634 (kW kvar) 162.86 114.93 121.78 92.95 121.84 93.07 406.48 300.95
  note: 692 --------A-------- --------B-------- --------C-------- ---V1--PQtotal---
      | V (pu deg.) 0.9871 -5.53 1.0519 -122.41 0.9780 116.00 1.0054 -3.94
      | Gen (kW kvar) 0.00 0.00 0.00 0.00 0.00 0.00 0.00 0.00
      | PQ load (kW kvar) 42.83 122.30 0.00 -0.00 125.48 27.20 168.31 149.50
      | Z shunt (kW kvar) 0.00 -0.00 -0.00 -0.00 0.00 -0.00 0.00 0.00
      |
      | -> 671 (kW kvar) -531.02 -121.99 -68.34 161.79 -416.10 -48.57 -1015.46 -8.77
      | -> 675 (kW kvar) 488.19 -0.30 68.34 -161.79 290.62 21.37 847.15 -140.72
  Anlges 692 : Display
  Complex to Magnitude-Angle : ComplexToMagnitudeAngle
  Complex to Magnitude-Angle2 : ComplexToMagnitudeAngle
  Complex to Magnitude-Angle3 : ComplexToMagnitudeAngle
  Multimeter : powerlib/Measurements/Multimeter  PhasorSimulation=off  OutputType=Complex  sel=[8 9 10]  L=20  Gain=[1 1 1]  yselected={'Uab: 692 D I','Ubc: 692 D I','Uca: 692 D I'};  PSBOutputType=1  PSBequivalent=0  AxesSetting=[0,0.1,-100,100]  Display=0  SavedBlockNames=-11
      settings: SourceProductBaseCode=MT,PS
  Multimeter1 : powerlib/Measurements/Multimeter  PhasorSimulation=off  OutputType=Complex  sel=[18 19 20]  L=20  Gain=[1 1 1]  yselected={'Iab: 692 D I','Ibc: 692 D I','Ica: 692 D I'};  PSBOutputType=1  PSBequivalent=0  AxesSetting=[0,0.1,-100,100]  Display=0  SavedBlockNames=-11
      settings: SourceProductBaseCode=MT,PS
  Multimeter2 : powerlib/Measurements/Multimeter  PhasorSimulation=off  OutputType=Complex  sel=[2 3 4]  L=20  Gain=[1 1 1]  yselected={'Uab: 671 D PQ','Ubc: 671 D PQ','Uca: 671 D PQ'};  PSBOutputType=1  PSBequivalent=0  AxesSetting=[0,0.1,-100,100]  Display=0  SavedBlockNames=-11
      settings: SourceProductBaseCode=MT,PS
  Multimeter3 : powerlib/Measurements/Multimeter  PhasorSimulation=off  OutputType=Complex  sel=[12 13 14]  L=20  Gain=[1 1 1]  yselected={'Iab: 671 D PQ','Ibc: 671 D PQ','Ica: 671 D PQ'};  PSBOutputType=1  PSBequivalent=0  AxesSetting=[0,0.1,-100,100]  Display=0  SavedBlockNames=-11
      settings: SourceProductBaseCode=MT,PS
  Multimeter4 : powerlib/Measurements/Multimeter  PhasorSimulation=off  OutputType=Complex  sel=1  L=20  Gain=1  yselected={'Ub: 611 I'};  PSBOutputType=1  PSBequivalent=0  AxesSetting=[0,0.1,-100,100]  Display=0  SavedBlockNames=-11
      settings: SourceProductBaseCode=MT,PS
  Multimeter5 : powerlib/Measurements/Multimeter  PhasorSimulation=off  OutputType=Complex  sel=11  L=20  Gain=1  yselected={'Ib: 611 I'};  PSBOutputType=1  PSBequivalent=0  AxesSetting=[0,0.1,-100,100]  Display=0  SavedBlockNames=-11
      settings: SourceProductBaseCode=MT,PS
  P 633->634 : Display
  P 692->675 : Display
  P Gen 632 : Display
  P_Load 611 I : Display
  P_Load 671 D PQ : Display
  P_Load 692 D I : Display
  Power (Phasor){,1..5} (6 alike) : powerlib_meascontrol/Measurements/Power (Phasor)
      settings: SourceProductBaseCode=MT,PS
  Q 633->634 : Display
  Q 692->675 : Display
  Q Gen 632 : Display
  Q_Load 611 I : Display
  Q_Load 671 D PQ : Display
  Q_Load 692 D I : Display
  V PG  692 : Display
  V PG 632 : Display
  V PG 633 : Display
  V->pu1 : Gain  Gain=1/(4160/sqrt(3)*sqrt(2))
  V->pu2 : Gain  Gain=1/(4160/sqrt(3)*sqrt(2))
  V->pu3 : Gain  Gain=1/(4160/sqrt(3)*sqrt(2))
  rad2deg : Gain  Gain=180/pi
  wires:
  [Iabc_692] -> Power (Phasor)1/2
  Power (Phasor)1/1 -> P 692->675/1
  Power (Phasor)1/2 -> Q 692->675/1
  [Vabc_692] -> Power (Phasor)1/1
  [Iabc_633] -> Power (Phasor)2/2
  Power (Phasor)2/1 -> P 633->634/1
  Power (Phasor)2/2 -> Q 633->634/1
  Complex to Magnitude-Angle2/1 -> V->pu1/1
  [Vabc_633] -> Power (Phasor)2/1, Complex to Magnitude-Angle2/1
  V->pu1/1 -> V PG 633/1
  [Iabc_632] -> Power (Phasor)3/2
  Power (Phasor)3/1 -> P Gen 632/1
  Power (Phasor)3/2 -> Q Gen 632/1
  Complex to Magnitude-Angle3/1 -> V->pu2/1
  [Vabc_632] -> Power (Phasor)3/1, Complex to Magnitude-Angle3/1
  V->pu2/1 -> V PG 632/1
  Multimeter/1 -> Power (Phasor)/1
  Multimeter1/1 -> Power (Phasor)/2
  Power (Phasor)/1 -> P_Load 692 D I/1
  Power (Phasor)/2 -> Q_Load 692 D I/1
  Multimeter2/1 -> Power (Phasor)4/1
  Multimeter3/1 -> Power (Phasor)4/2
  Power (Phasor)4/1 -> P_Load 671 D PQ/1
  Power (Phasor)4/2 -> Q_Load 671 D PQ/1
  Complex to Magnitude-Angle/1 -> V->pu3/1
  [Vabc_692] -> Complex to Magnitude-Angle/1
  Complex to Magnitude-Angle/2 -> rad2deg/1
  rad2deg/1 -> Anlges 692/1
  Multimeter4/1 -> Power (Phasor)5/1
  Multimeter5/1 -> Power (Phasor)5/2
  Power (Phasor)5/1 -> P_Load 611 I/1
  Power (Phasor)5/2 -> Q_Load 611 I/1
  V->pu3/1 -> V PG  692/1
